simulink model "System_Model"  (R2026b)
settings: Solver=VariableStepAuto
InitFcn:
  | params;
values from neighbouring files (symbols this model uses):
  dt = 1/30    (= 0.0333333333333)    [system_params.m]
  q0 = [0; -pi/2; pi/2; -pi/2; -pi/2; 0]    [system_params.m]
undefined symbols (not defined in the file or in its folder): DiscIntNeverNeededParam
libraries: robotmaniplib x2
settings Model: Creator=youss  LastModifiedBy=youss

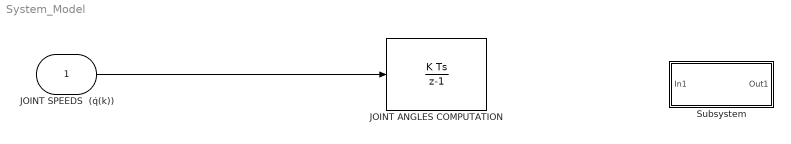
== system System_Model ==
  JOINT SPEEDS  (q̇(k)) : Inport
  JOINT ANGLES COMPUTATION : DiscreteIntegrator  InitialCondition=q0  SampleTime=dt  ICPrevOutput=DiscIntNeverNeededParam  ICPrevScaledInput=DiscIntNeverNeededParam
  Subsystem : Subsystem
  wires:
  JOINT SPEEDS  (q̇(k))/1 -> JOINT ANGLES COMPUTATION/1

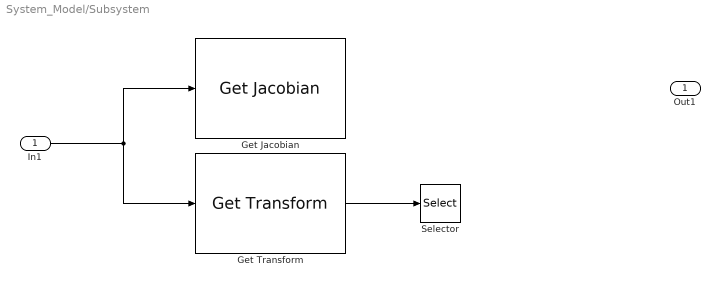
== system System_Model/Subsystem ==
  In1 : Inport
  Get Jacobian : robotmaniplib/Get Jacobian  RigidBodyTree=ur5  EndEffector=camera  SimulateUsing=Interpreted execution
  Get Transform : robotmaniplib/Get Transform  RigidBodyTree=ur5  SourceBody=base  TargetBody=camera  SimulateUsing=Interpreted execution
  Selector : Selector  NumberOfDimensions=2  InputPortWidth=3  IndexOptions=Index vector (dialog),Index vector (dialog)  Indices=[1 2 3],[1 2 3]  OutputSizes=1,1
  Out1 : Outport
  wires:
  In1/1 -> Get Transform/1, Get Jacobian/1
  Get Transform/1 -> Selector/1
